simulink model "pv_model_F8_inter_string_short"  (R2025b)
settings: Solver=FixedStepDiscrete  StartTime=0.0  StopTime=86400  FixedStep=1  RelTol=1e-3
undefined symbols (not defined in the file): RF8, Rload_day, timef8, Ts_Control, Ts_Power, Vnom_dc
libraries: spsPVArrayLib x22, spsCurrentMeasurementLib x11, spsSeriesRLCBranchLib x2, spsPVarrayModel x2, spsMeanLib x2, spsIdealSwitchLib x1, spsVoltageMeasurementLib x1, spspowerguiLib x1
settings Model: Creator=edgar  LastModifiedBy=edgar
settings DataIOCC: LimitDataPoints=on  SaveFormat=Array  DSMLogging=off  ReturnWorkspaceOutputs=off
settings DebuggingCC: AlgebraicLoopMsg=none  SolverPrmCheckMsg=warning  FcnCallInpInsideContextMsg=warning  StateNameClashWarn=warning  SFUnexpectedBacktrackingDiag=warning  SFNoUnconditionalDefaultTransitionDiag=warning  SFExecutionAtInitializationDiag=none
settings ModelReferenceCC: EnableRefExpFcnMdlSchedulingChecks=on  PropagateSignalLabelsOutOfModel=off

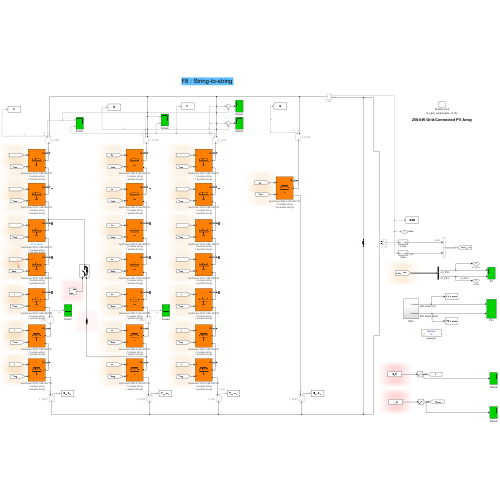
[thumbnail: Simulink's stored preview of the top-level diagram]
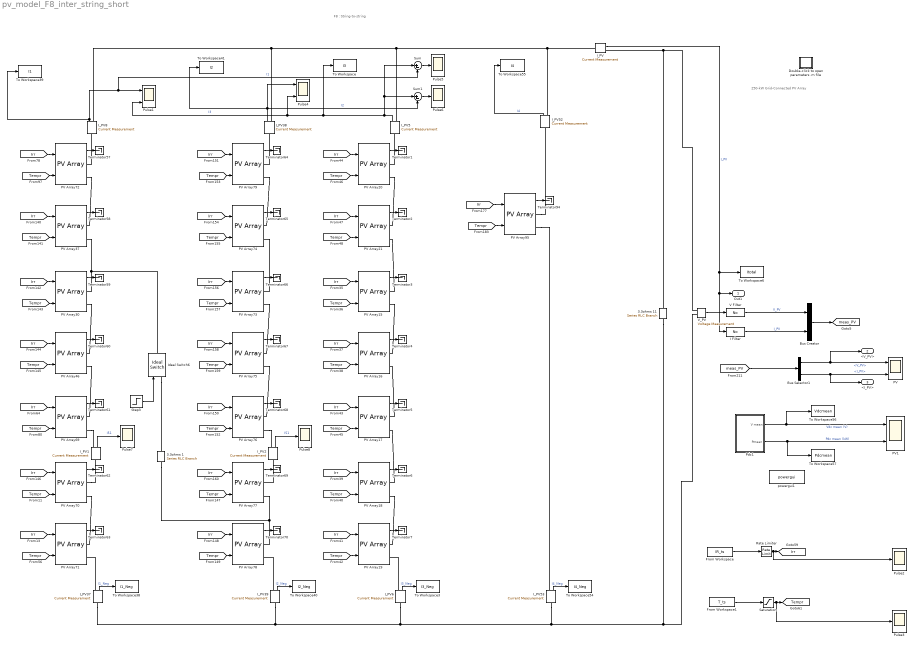
== system pv_model_F8_inter_string_short ==
  note: F8 : String-to-string
  note: 250-kW Grid-Connected PV Array
  3.3ohms 1 : spsSeriesRLCBranchLib/Series RLC Branch  LConnTagsString=__new0  RConnTagsString=__new0  BranchType=R  Resistance=RF8  Inductance=[]  SetiL0=off  InitialCurrent=0  Capacitance=[]  Setx0=off  InitialVoltage=0  Measurements=None
  3.3ohms 11 : spsSeriesRLCBranchLib/Series RLC Branch  LConnTagsString=__new0  RConnTagsString=__new0  BranchType=R  Resistance=Rload_day  Inductance=[]  SetiL0=off  InitialCurrent=0  Capacitance=[]  Setx0=off  InitialVoltage=0  Measurements=None
  Bus Creator : BusCreator  Inputs=2
  Bus Selector1 : BusSelector  OutputSignals=V_PV,I_PV
  Double-click to open parameters .m file : Subsystem
      settings: OpenFcn=open('power_PVarray_250kW_param.m')
  From Workspace : FromWorkspace  VariableName=IR_ts  SampleTime=1
  From Workspace1 : FromWorkspace  VariableName=T_ts  SampleTime=1
  I Filter : spsPVarrayModel/No  SystemSampleTime=-1  VariantControl=Variant1  VariantActivationTime=update diagram  EmptyChoice=off  PassThrough=off  PassThroughVariantControl=(default)  EmptyChoiceVariantControl=(default)  AllowFlexibleInterface=on  Latency=0  AutoFrameSizeCalculation=off
  I_PV{,1..2,5..6,8,37..39,52..53} (11 alike) : spsCurrentMeasurementLib/Current Measurement  PhasorSimulation=off  OutputType=Complex  PSBequivalent=0
  Ideal Switch6 : spsIdealSwitchLib/Ideal Switch  Ron=0.001  Lon=0  IC=0  Rs=1e4  Cs=1e-10  Measurements=off
  PV : Scope  NumInputPorts=2
      settings: TimeSpan=1.5  ActiveDisplayYMinimum=-71.710124808649638  ActiveDisplayYMaximum=645.39088592996507  DataLoggingDecimation=10  DataLoggingSaveFormat=Array
  PV Array{15..21,30,37,46,69..79} (21 alike) : spsPVArrayLib/PV Array  Npar=1  Nser=1  PlotType=array @ 1000 W/m2 & specified temperatures  S_vec="[ 1000  500  100 ]"  Temp_C_vec="[ 45 25  ]"  ModuleName=SunPower SPR-415E-WHT-D  PlotWhenSelected=off  Pm=414.801  Ncell=128  Voc=85.3  Isc=6.09  Vm=72.9  Im=5.69  beta_Voc_pc=-0.229  alpha_Isc_pc=0.030706  beta_Voc=-0.19534  alpha_Isc=0.00187  IL=6.0978  I0=7.1698e-13  nI=0.87223  Rsh=419.7781  Rs=0.53711  RobustModel=off  RobustCellTemperature=313.3991  BAL=off  Tc=1e-6  Tfilter=5e-5
      settings: AttributesFormatString=|
      | %<ModuleName>
      | %<Nser>-module string
      | %<Npar> parallel strings
  PV Array95 : spsPVArrayLib/PV Array  Npar=19  Nser=7  PlotType=array @ 1000 W/m2 & specified temperatures  S_vec="[ 1000  500  100 ]"  Temp_C_vec="[ 45 25  ]"  ModuleName=SunPower SPR-415E-WHT-D  PlotWhenSelected=off  Pm=414.801  Ncell=128  Voc=85.3  Isc=6.09  Vm=72.9  Im=5.69  beta_Voc_pc=-0.229  alpha_Isc_pc=0.030706  beta_Voc=-0.19534  alpha_Isc=0.00187  IL=6.0978  I0=7.1698e-13  nI=0.87223  Rsh=419.7781  Rs=0.53711  RobustModel=off  RobustCellTemperature=313.3991  BAL=off  Tc=1e-6  Tfilter=5e-5
      settings: AttributesFormatString=|
      | %<ModuleName>
      | %<Nser>-module string
      | %<Npar> parallel strings
  PV1 : Scope  NumInputPorts=2
      settings: TimeSpan=1.5  ActiveDisplayYMinimum=208.04916  ActiveDisplayYMaximum=527.55759  DataLoggingDecimation=10  DataLoggingVariableName=ScopeData15  DataLoggingSaveFormat=Array
  Pdc1 : Subsystem
  Pulse1 : Scope  NumInputPorts=2
      settings: TimeSpan=1.5  ActiveDisplayYMinimum=3.7545284060958322  ActiveDisplayYMaximum=3.8181914115261564  DataLoggingDecimation=10  DataLoggingSaveFormat=Array
  Pulse{2..3,5..8} (6 alike) : Scope
      Pulse2 settings: TimeSpan=1.5  ActiveDisplayYMinimum=-118.4528917980434  ActiveDisplayYMaximum=1066.0760261823907  DataLoggingDecimation=10  DataLoggingVariableName=ScopeData12  DataLoggingSaveFormat=Array
      Pulse3 settings: TimeSpan=1.5  ActiveDisplayYMinimum=14.376202367904177  ActiveDisplayYMaximum=30.614178688862403  DataLoggingDecimation=10  DataLoggingVariableName=ScopeData13  DataLoggingSaveFormat=Array
      Pulse5 settings: TimeSpan=1.5  ActiveDisplayYMinimum=-3.696460297871798E-6  ActiveDisplayYMaximum=3.3003296172496625E-5  DataLoggingDecimation=10  DataLoggingVariableName=ScopeData3  DataLoggingSaveFormat=Array
      Pulse6 settings: TimeSpan=1.5  ActiveDisplayYMinimum=-6.600659229603602E-6  ActiveDisplayYMaximum=7.3929205903359476E-7  DataLoggingDecimation=10  DataLoggingVariableName=ScopeData4  DataLoggingSaveFormat=Array
      Pulse7 settings: TimeSpan=1.5  ActiveDisplayYMinimum=-118.4528917980434  ActiveDisplayYMaximum=1066.0760261823907  DataLoggingDecimation=10  DataLoggingVariableName=ScopeData5  DataLoggingSaveFormat=Array
      Pulse8 settings: TimeSpan=1.5  ActiveDisplayYMinimum=-118.4528917980434  ActiveDisplayYMaximum=1066.0760261823907  DataLoggingDecimation=10  DataLoggingVariableName=ScopeData6  DataLoggingSaveFormat=Array
  Pulse4 : Scope  NumInputPorts=2
      settings: TimeSpan=1.5  ActiveDisplayYMinimum=3.5912796995552028  ActiveDisplayYMaximum=4.1749700186901455  DataLoggingDecimation=10  DataLoggingVariableName=ScopeData2  DataLoggingSaveFormat=Array
  Rate Limiter : RateLimiter  RisingSlewLimit=6000  FallingSlewLimit=-6000  SampleTimeMode=inherited  InitialCondition=1000
  Saturation : Saturate  UpperLimit=55  LowerLimit=5
  Step3 : Step  Time=timef8  SampleTime=Ts_Power
  Sum : Sum  Inputs=|+-
  Sum1 : Sum  Inputs=|+-
  Terminator{1..7,57..70,94} (22 alike) : Terminator
  To Workspace : ToWorkspace  VariableName=I3  SampleTime=-1
      settings: Save2DSignal=2-D array (concatenate along first dimension)
  To Workspace3 : ToWorkspace  VariableName=I3_Neg  SampleTime=-1
      settings: Save2DSignal=2-D array (concatenate along first dimension)
  To Workspace38 : ToWorkspace  VariableName=I1_Neg  SampleTime=-1
      settings: Save2DSignal=2-D array (concatenate along first dimension)
  To Workspace39 : ToWorkspace  VariableName=I1  SampleTime=-1
      settings: Save2DSignal=2-D array (concatenate along first dimension)
  To Workspace40 : ToWorkspace  VariableName=I2_Neg  SampleTime=-1
      settings: Save2DSignal=2-D array (concatenate along first dimension)
  To Workspace41 : ToWorkspace  VariableName=I2  SampleTime=-1
      settings: Save2DSignal=2-D array (concatenate along first dimension)
  To Workspace54 : ToWorkspace  VariableName=I4_Neg  SampleTime=-1
      settings: Save2DSignal=2-D array (concatenate along first dimension)
  To Workspace55 : ToWorkspace  VariableName=I4  SampleTime=-1
      settings: Save2DSignal=2-D array (concatenate along first dimension)
  To Workspace56 : ToWorkspace  VariableName=Vdcmean  SampleTime=-1
      settings: Save2DSignal=2-D array (concatenate along first dimension)
  To Workspace57 : ToWorkspace  VariableName=Pdcmean  SampleTime=-1
      settings: Save2DSignal=2-D array (concatenate along first dimension)
  To Workspace6 : ToWorkspace  VariableName=Itotal  SampleTime=-1
      settings: Save2DSignal=2-D array (concatenate along first dimension)
  V Filter : spsPVarrayModel/No  SystemSampleTime=-1  VariantControl=Variant1  VariantActivationTime=update diagram  EmptyChoice=off  PassThrough=off  PassThroughVariantControl=(default)  EmptyChoiceVariantControl=(default)  AllowFlexibleInterface=on  Latency=0  AutoFrameSizeCalculation=off
  V_PV : spsVoltageMeasurementLib/Voltage Measurement  PhasorSimulation=off  OutputType=Complex  PSBequivalent=0
  powergui1 : spspowerguiLib/powergui  Priority=1  SimulationMode=Discrete  SampleTime=Ts_Power  frequency=60  Iterations=50  frequencyindice=0  Pbase=100e6  ErrMax=1e-4  UnitsV=kV  UnitsW=MW  buscounter=0  FunctionMessages=off  echomessages=off  EnableUseOfTLC=off  CurrentSourceSwitches=off  DisableSnubberDevices=off  DisableRonSwitches=off  DisableVfSwitches=off  DisplayEquations=off  AutomaticDiscreteSolvers=off  SolverType=Tustin  Interpol=off  ExternalGateDelay=off  methode=off  Ts=0  x0status=blocks  SPID=off  SwTol=0  HookPort=off  NonlinearTolerance=1e-4  nMaxIteration=100  ContinueOnMaxIteration=off  RestoreLinks=warning  ResistiveCurrentMeasurement=off  Frange=[0:2:500]  Ylog=off  Xlog=on  ShowGrid=off  save=off  variable=ZData  structure=VaIa_Grid  ZoomFFT=off  StartTime=1.4  cycles=3  DisplayStyle=1  fundamental=60  FreqAxis=on  MaxFrequency=5000  frequencyindicesteady=1  RmsSteady=1  display=off
  Out1 : Outport  SignalName=totalc  VectorParamsAs1DForOutWhenUnconnected=off
  <V_PV> : Outport  Port=2
  <I_PV> : Outport  Port=3
  tag scope: Irr=global, Tempr=global, meas_PV=global
  wires:
  Sum1/1 -> Pulse6/1
  PV Array71/1 -> Terminator63/1
  [Irr] -> PV Array78/1
  [Irr] -> PV Array46/1
  [Irr] -> PV Array95/1
  PV Array69/1 -> Terminator61/1
  [Tempr] -> PV Array46/2
  Bus Selector1/2 -> <I_PV>/1, PV/2  "<I_PV>"
  [Tempr] -> PV Array69/2
  PV Array79/1 -> Terminator64/1
  [Irr] -> PV Array72/1
  From Workspace1/1 -> Saturation/1
  [Tempr] -> PV Array95/2
  [Tempr] -> PV Array75/2
  [Irr] -> PV Array76/1
  [Irr] -> PV Array75/1
  PV Array77/1 -> Terminator69/1
  [Tempr] -> PV Array74/2
  [Tempr] -> PV Array72/2
  [Tempr] -> PV Array79/2
  Pdc1/1(V mean) -> To Workspace56/1, PV1/1  "Vdc mean (V)"
  Rate Limiter/1 -> Pulse2/1, [Irr]
  [Tempr] -> PV Array30/2
  Step3/1 -> Ideal Switch6/1
  I_PV2/1 -> Pulse8/1  "I51"
  PV Array73/1 -> Terminator66/1
  [Irr] -> PV Array77/1
  [Tempr] -> PV Array77/2
  [Irr] -> PV Array70/1
  I_PV38/1 -> To Workspace41/1, Sum1/2, Pulse4/1  "I2"
  [Irr] -> PV Array30/1
  [Irr] -> PV Array37/1
  PV Array37/1 -> Terminator58/1
  PV Array95/1 -> Terminator94/1
  [Irr] -> PV Array79/1
  PV Array78/1 -> Terminator70/1
  Pdc1/2(Pmean) -> To Workspace57/1, PV1/2  "Pdc mean (kW)"
  [Tempr] -> PV Array73/2
  I_PV8/1 -> Sum/2, Pulse1/1, To Workspace39/1  "I1"
  PV Array74/1 -> Terminator65/1
  I_PV/1 -> To Workspace6/1, Out1/1, I Filter/1  "I_PV"
  PV Array75/1 -> Terminator67/1
  I_PV1/1 -> Pulse7/1  "I51"
  V_PV/1 -> V Filter/1
  [Irr] -> PV Array16/1
  PV Array19/1 -> Terminator7/1
  PV Array15/1 -> Terminator3/1
  PV Array20/1 -> Terminator1/1
  PV Array21/1 -> Terminator2/1
  [Tempr] -> PV Array16/2
  [Irr] -> PV Array19/1
  PV Array17/1 -> Terminator5/1
  PV Array16/1 -> Terminator4/1
  ? -> ?  "I2"
  [Tempr] -> PV Array21/2
  [Tempr] -> PV Array17/2
  [Tempr] -> PV Array20/2
  [Irr] -> PV Array17/1
  [Irr] -> PV Array18/1
  [Irr] -> PV Array21/1
  I_PV37/1 -> To Workspace38/1  "I1_Neg"
  I_PV52/1 -> To Workspace55/1  "I4"
  I_PV53/1 -> To Workspace54/1  "I4_Neg"
  I_PV39/1 -> To Workspace40/1  "I2_Neg"
  PV Array46/1 -> Terminator60/1
  [Irr] -> PV Array71/1
  [meas_PV] -> Bus Selector1/1
  [Irr] -> PV Array15/1
  [Irr] -> PV Array69/1
  [Tempr] -> PV Array70/2
  [Tempr] -> PV Array15/2
  [Tempr] -> PV Array78/2
  From Workspace/1 -> Rate Limiter/1
  Bus Creator/1 -> [meas_PV]
  [Irr] -> PV Array73/1
  I Filter/1 -> Bus Creator/2  "I_PV"
  PV Array30/1 -> Terminator59/1
  [Tempr] -> PV Array71/2
  Saturation/1 -> Pulse3/1, [Tempr]
  [Irr] -> PV Array74/1
  [Tempr] -> PV Array76/2
  [Irr] -> PV Array20/1
  PV Array76/1 -> Terminator68/1
  [Tempr] -> PV Array18/2
  Bus Selector1/1 -> PV/1, <V_PV>/1  "<V_PV>"
  [Tempr] -> PV Array37/2
  I_PV6/1 -> To Workspace3/1  "I3_Neg"
  PV Array70/1 -> Terminator62/1
  Sum/1 -> Pulse5/1
  PV Array72/1 -> Terminator57/1
  [Tempr] -> PV Array19/2
  V Filter/1 -> Bus Creator/1  "V_PV"
  PV Array18/1 -> Terminator6/1
  I_PV5/1 -> Pulse1/2, Pulse4/2, To Workspace/1, Sum1/1, Sum/1  "I3"
  connections:
  I_PV/RConn1 -- V_PV/LConn1 -- 3.3ohms 11/LConn1
  Ideal Switch6/RConn1 -- PV Array30/RConn1 -- PV Array37/RConn2
  I_PV52/RConn1 -- I_PV5/RConn1 -- I_PV8/RConn1 -- I_PV38/RConn1 -- I_PV/LConn1
  V_PV/LConn2 -- 3.3ohms 11/RConn1 -- I_PV6/LConn1 -- I_PV37/LConn1 -- I_PV39/LConn1 -- I_PV53/LConn1
  PV Array77/RConn2 -- 3.3ohms 1/LConn1 -- PV Array78/RConn1
  PV Array69/RConn2 -- I_PV1/RConn1
  PV Array30/RConn2 -- PV Array46/RConn1
  I_PV39/RConn1 -- PV Array78/RConn2
  PV Array73/RConn2 -- PV Array75/RConn1
  PV Array72/RConn2 -- PV Array37/RConn1
  PV Array95/RConn2 -- I_PV53/RConn1
  PV Array75/RConn2 -- PV Array76/RConn1
  I_PV2/LConn1 -- PV Array77/RConn1
  PV Array20/RConn1 -- I_PV5/LConn1
  PV Array18/RConn1 -- PV Array17/RConn2
  I_PV6/RConn1 -- PV Array19/RConn2
  PV Array15/RConn1 -- PV Array21/RConn2
  Ideal Switch6/LConn1 -- 3.3ohms 1/RConn1
  PV Array20/RConn2 -- PV Array21/RConn1
  PV Array70/RConn1 -- I_PV1/LConn1
  PV Array17/RConn1 -- PV Array16/RConn2
  PV Array95/RConn1 -- I_PV52/LConn1
  PV Array18/RConn2 -- PV Array19/RConn1
  I_PV37/RConn1 -- PV Array71/RConn2
  PV Array46/RConn2 -- PV Array69/RConn1
  PV Array72/RConn1 -- I_PV8/LConn1
  PV Array79/RConn2 -- PV Array74/RConn1
  PV Array74/RConn2 -- PV Array73/RConn1
  PV Array76/RConn2 -- I_PV2/RConn1
  PV Array79/RConn1 -- I_PV38/LConn1
  PV Array15/RConn2 -- PV Array16/RConn1
  PV Array70/RConn2 -- PV Array71/RConn1

== system pv_model_F8_inter_string_short/Double-click to open parameters .m file ==

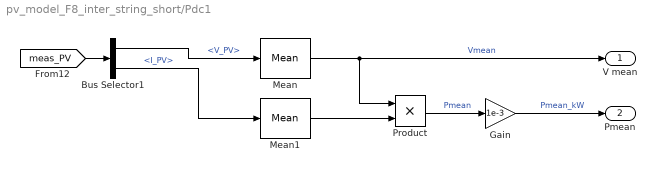
== system pv_model_F8_inter_string_short/Pdc1 ==
  Bus Selector1 : BusSelector  OutputSignals=V_PV,I_PV
  Gain : Gain  Gain=1e-3
  Mean : spsMeanLib/Mean  Freq=Fnom  Vinit=Vnom_dc/2  Ts=Ts_Control
  Mean1 : spsMeanLib/Mean  Freq=Fnom  Vinit=0  Ts=Ts_Control
  Product : Product
  V mean : Outport  VectorParamsAs1DForOutWhenUnconnected=off
  Pmean : Outport  Port=2  VectorParamsAs1DForOutWhenUnconnected=off
  wires:
  Mean/1 -> V mean/1, Product/1  "Vmean"
  Mean1/1 -> Product/2
  Product/1 -> Gain/1  "Pmean"
  Gain/1 -> Pmean/1  "Pmean_kW"
  Bus Selector1/1 -> Mean/1  "<V_PV>"
  Bus Selector1/2 -> Mean1/1  "<I_PV>"
  [meas_PV] -> Bus Selector1/1
